simulink model "sim_CS1B_linear"  (R2025b)
settings: Solver=ode45  StartTime=0.0  StopTime=Tsim  MaxStep=ts  RelTol=1e-6
values from neighbouring files (symbols this model uses):
  Ac = [0, 0, 1, 0 ... (first row only)    [qube_model.m]
  Bc = [0; 0; b*kv/Delta0; c*kv/Delta0]    [qube_model.m]
  step_time = 1    [design_and_simulate_CS1B.m]    (also in params_CS1B.m)
  theta_step = deg2rad(45)    [design_and_simulate_CS1B.m]    (also in params_CS1B.m = 0.785398163397)
  ts = 1/1000    (= 0.001)    [Hardware_settings.m]    (also in qube_model.m)
  x0 = zeros(4,1)    [design_and_simulate_CS1B.m]    (also in params_CS1B.m = [0; 0; 0; 0])
settings Model: Creator=jaylen  LastModifiedBy=jaylen
settings DataIOCC: SaveOutput=off  SaveTime=off

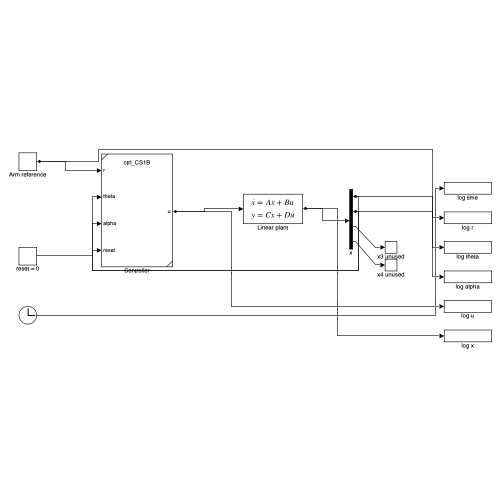
[thumbnail: Simulink's stored preview of the top-level diagram]
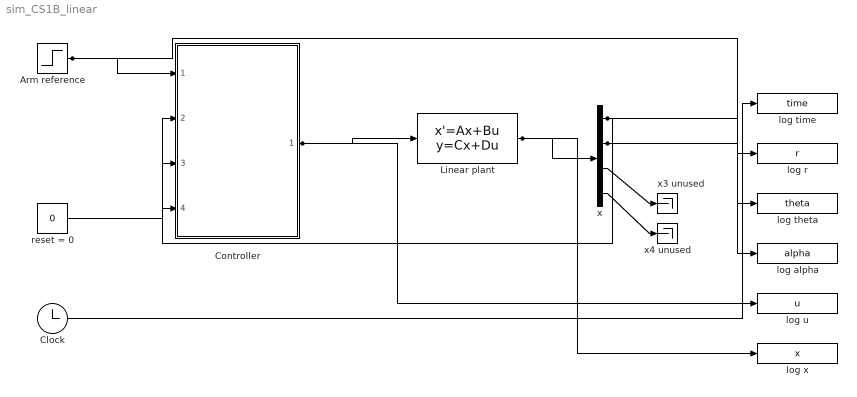
== system sim_CS1B_linear ==
  Arm reference : Step  Time=step_time  After=theta_step  SampleTime=ts
  Clock : Clock
  Controller : Subsystem  ReferencedSubsystem=ctrl_CS1B
  Linear plant : StateSpace  A=Ac  B=Bc  C=eye(4)  D=zeros(4,1)  InitialCondition=x0
  log alpha : ToWorkspace  VariableName=alpha  SampleTime=ts
  log r : ToWorkspace  VariableName=r  SampleTime=ts
  log theta : ToWorkspace  VariableName=theta  SampleTime=ts
  log time : ToWorkspace  VariableName=time  SampleTime=ts
  log u : ToWorkspace  VariableName=u  SampleTime=ts
  log x : ToWorkspace  VariableName=x  SampleTime=ts
  reset = 0 : Constant  Value=0
  x : Demux
  x3 unused : Terminator
  x4 unused : Terminator
  wires:
  Linear plant/1 -> x/1, log x/1
  Controller/1 -> Linear plant/1, log u/1
  Arm reference/1 -> Controller/1, log r/1
  x/1 -> Controller/2, log theta/1
  x/2 -> Controller/3, log alpha/1
  reset = 0/1 -> Controller/4
  x/3 -> x3 unused/1
  x/4 -> x4 unused/1
  Clock/1 -> log time/1
